simulink library "lib_TerCtrl_NoTC"  (R2026a)
settings: Solver=VariableStepAuto
undefined symbols (not defined in the file): buses_lf, Ps_lf, Qs_lf, vs_lf
settings Model: Creator=atomas  LastModifiedBy=atomas

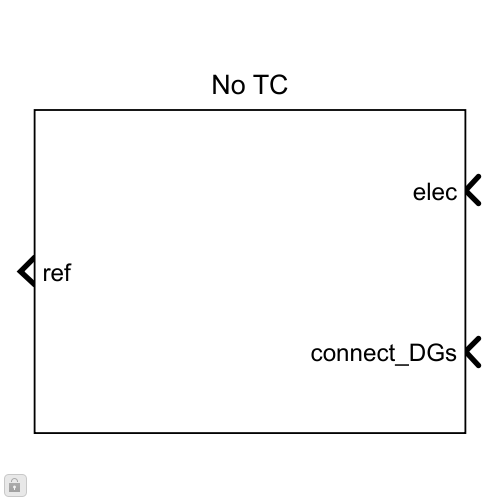
[thumbnail: Simulink's stored preview of the top-level diagram]
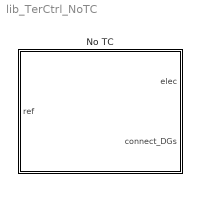
== system lib_TerCtrl_NoTC ==
  No TC : Subsystem  VariantControl=No TC

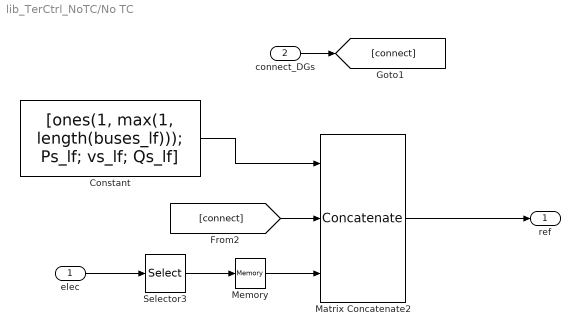
== system lib_TerCtrl_NoTC/No TC ==
  elec : Inport
  connect_DGs : Inport  Port=2
  Constant : Constant  Value=[ones(1, max(1, length(buses_lf))); Ps_lf; vs_lf; Qs_lf]  VectorParams1D=off
  Matrix Concatenate2 : Concatenate  NumInputs=3  Mode=Multidimensional array
  Memory : Memory  InitialCondition=1
  Selector3 : Selector  NumberOfDimensions=2  InputPortWidth=3  IndexOptions=Index vector (dialog),Select all  Indices=6,1  OutputSizes=1,1
  ref : Outport
  wires:
  Matrix Concatenate2/1 -> ref/1
  connect_DGs/1 -> [connect]
  [connect] -> Matrix Concatenate2/2
  Selector3/1 -> Memory/1
  elec/1 -> Selector3/1
  Constant/1 -> Matrix Concatenate2/1
  Memory/1 -> Matrix Concatenate2/3
